simulink model "ekf_pmsm"  (R2026a)
settings: Solver=FixedStepDiscrete  StartTime=0  StopTime=1.5  FixedStep=1/15000
PreLoadFcn:
  | addpath('F:\code\foc\Doc\matlab');
StartFcn:
  | clear sl_if_ctrl sl_ekf sl_pmsm_meas;
libraries: fl_lib x9, nesl_utility x9, ee_lib x1
Description:
  | ATK-BL57H95D20E：Simscape Electrical PMSM + I/F + EKF
settings Model: Creator=15403  LastModifiedBy=15403

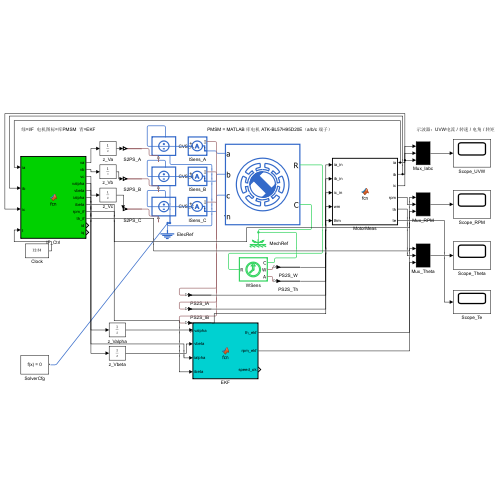
[thumbnail: Simulink's stored preview of the top-level diagram]
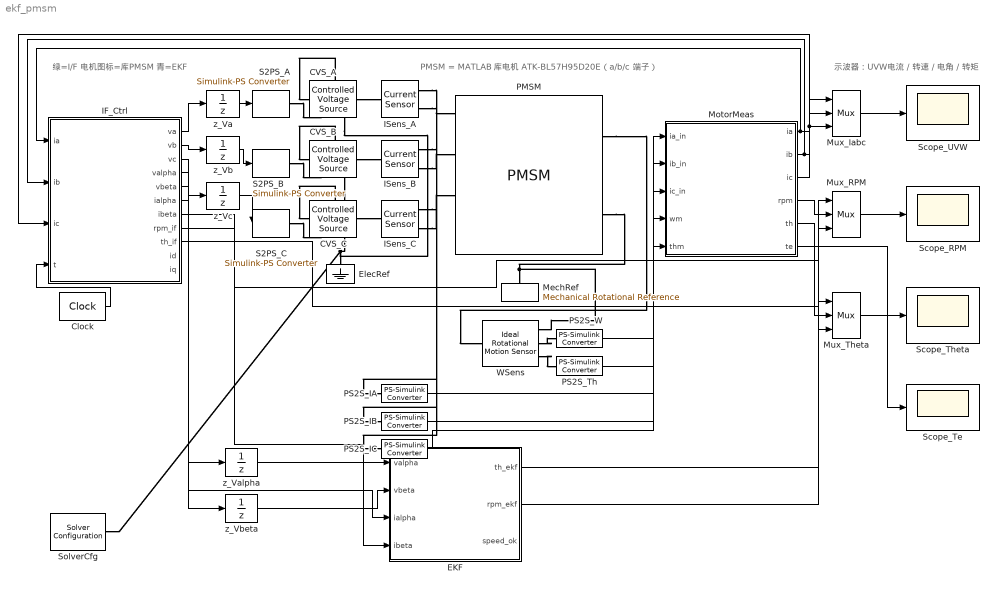
== system ekf_pmsm ==
  note: PMSM = MATLAB 库电机 ATK-BL57H95D20E（a/b/c 端子）
  note: 示波器：UVW电流 / 转速 / 电角 / 转矩
  note: 绿=I/F 电机图标=库PMSM 青=EKF
  CVS_A : fl_lib/Electrical/Electrical Sources/Controlled Voltage Source
  CVS_B : fl_lib/Electrical/Electrical Sources/Controlled Voltage Source
  CVS_C : fl_lib/Electrical/Electrical Sources/Controlled Voltage Source
  Clock : DigitalClock  SampleTime=1/15000
  EKF : MATLAB Function  TreatAsAtomicUnit=on
  ElecRef : fl_lib/Electrical/Electrical Elements/Electrical Reference
  IF_Ctrl : MATLAB Function  TreatAsAtomicUnit=on
  ISens_A : fl_lib/Electrical/Electrical Sensors/Current Sensor
  ISens_B : fl_lib/Electrical/Electrical Sensors/Current Sensor
  ISens_C : fl_lib/Electrical/Electrical Sensors/Current Sensor
  MechRef : fl_lib/Mechanical/Rotational Elements/Mechanical Rotational Reference
  MotorMeas : MATLAB Function  TreatAsAtomicUnit=on
  Mux_Iabc : Mux  Inputs=3
  Mux_RPM : Mux  Inputs=3
  Mux_Theta : Mux  Inputs=3
  PMSM : ee_lib/Electromechanical/Permanent Magnet/PMSM  port_option=ee.enum.threePhasePort.expanded  winding_type=ee.enum.electromech.statorconfiguration.wye  machine_param=ee.enum.pmsm.parameterization.constant  nPolePairs=2  pmflux_param=ee.enum.pmflux.fluxlinkage  pm_flux_linkage=0.02573 Wb  torque_constant=0.18 N*m/A  back_emf_constant=0.18 V*s/rad  stator_param=ee.enum.statorparam.LdLqL0  Ld=0.0008 H  Lq=0.0008 H  idVec=[-200, 0, 200] A  iqVec=[-200, 0, 200] A  LdMatrix=0.0002 * ones(3, 3) H  LqMatrix=0.0002 * ones(3, 3) H  PmMatrix=0.1 * ones(3, 3) Wb  ktMatrix=0.18 * ones(3, 3) N*m/A  keMatrix=0.18 * ones(3, 3) V*s/rad  L0=0.0008 H  Ls=0.0002 H  Lm=-0.00002 H  Ms=0.00002 H  Rs=0.4 Ohm  zero_sequence=ee.enum.park.zerosequence.include  axes_param=ee.enum.rotorangle.daxis  loss_param=ee.enum.ironloss.none  losses_oc=[0, 0, 0] W  losses_sc=[0, 0, 0] W  f_losses=60 Hz  Isc_losses=95 A  J=2.1e-05 kg*m^2  lam=5.25e-05 N*m*s/rad  i_d_specify=off  i_d_priority=None  i_d=0 A  i_d_nominal_specify=off  i_d_nominal_value=1  i_d_nominal_unit=A  i_q_specify=off  i_q_priority=None  i_q=0 A  i_q_nominal_specify=off  i_q_nominal_value=1  i_q_nominal_unit=A  torque_specify=off  torque_priority=None  torque=0 N*m  torque_nominal_specify=off  torque_nominal_value=1  torque_nominal_unit=N*m  angular_velocity_specify=off  angular_velocity_priority=High  angular_velocity=0 rpm  angular_velocity_nominal_specify=off  angular_velocity_nominal_value=1  angular_velocity_nominal_unit=rpm  angular_position_specify=off  angular_position_priority=High  angular_position=0 deg  angular_position_nominal_specify=off  angular_position_nominal_value=1  angular_position_nominal_unit=deg  alpha=3.93e-3 1/K  alpha_flux=-0.001 1/K  Tmeas=298.15 K  stator_thermal_mass=100 J/K  rotor_thermal_mass=200 J/K  Rm_percent_rotor=90  Rd_percent_rotor=30  temperatureA_specify=off  temperatureA_priority=High  temperatureA=25 degC  temperatureA_nominal_specify=off  temperatureA_nominal_value=1  temperatureA_nominal_unit=degC  temperatureB_specify=off  temperatureB_priority=High  temperatureB=25 degC  temperatureB_nominal_specify=off  temperatureB_nominal_value=1  temperatureB_nominal_unit=degC  temperatureC_specify=off  temperatureC_priority=High  temperatureC=25 degC  temperatureC_nominal_specify=off  temperatureC_nominal_value=1  temperatureC_nominal_unit=degC  temperatureR_specify=off  temperatureR_priority=High  temperatureR=25 degC  temperatureR_nominal_specify=off  temperatureR_nominal_value=1  temperatureR_nominal_unit=degC
  PS2S_IA : nesl_utility/PS-Simulink Converter  PhysicalDomain=network_engine_domain  SubClassName=ps_output  LeftPortType=input  RightPortType=output  PseudoPeriodic=off  Frequencies=[]  VectorFormat=inherit  Unit=A  AffineConversion=off
  PS2S_IB : nesl_utility/PS-Simulink Converter  PhysicalDomain=network_engine_domain  SubClassName=ps_output  LeftPortType=input  RightPortType=output  PseudoPeriodic=off  Frequencies=[]  VectorFormat=inherit  Unit=A  AffineConversion=off
  PS2S_IC : nesl_utility/PS-Simulink Converter  PhysicalDomain=network_engine_domain  SubClassName=ps_output  LeftPortType=input  RightPortType=output  PseudoPeriodic=off  Frequencies=[]  VectorFormat=inherit  Unit=A  AffineConversion=off
  PS2S_Th : nesl_utility/PS-Simulink Converter  PhysicalDomain=network_engine_domain  SubClassName=ps_output  LeftPortType=input  RightPortType=output  PseudoPeriodic=off  Frequencies=[]  VectorFormat=inherit  Unit=rad  AffineConversion=off
  PS2S_W : nesl_utility/PS-Simulink Converter  PhysicalDomain=network_engine_domain  SubClassName=ps_output  LeftPortType=input  RightPortType=output  PseudoPeriodic=off  Frequencies=[]  VectorFormat=inherit  Unit=rad/s  AffineConversion=off
  S2PS_A : nesl_utility/Simulink-PS Converter  PhysicalDomain=network_engine_domain  SubClassName=ps_input  LeftPortType=input  RightPortType=output  PseudoPeriodic=off  Frequencies=[]  NoiseDistribution=none  NoiseParameters=[]  Unit=V  AffineConversion=off  FilteringAndDerivatives=provide  SimscapeFilterOrder=1  InputFilterTimeConstant=0.001  UdotUserProvided=0
  S2PS_B : nesl_utility/Simulink-PS Converter  PhysicalDomain=network_engine_domain  SubClassName=ps_input  LeftPortType=input  RightPortType=output  PseudoPeriodic=off  Frequencies=[]  NoiseDistribution=none  NoiseParameters=[]  Unit=V  AffineConversion=off  FilteringAndDerivatives=provide  SimscapeFilterOrder=1  InputFilterTimeConstant=0.001  UdotUserProvided=0
  S2PS_C : nesl_utility/Simulink-PS Converter  PhysicalDomain=network_engine_domain  SubClassName=ps_input  LeftPortType=input  RightPortType=output  PseudoPeriodic=off  Frequencies=[]  NoiseDistribution=none  NoiseParameters=[]  Unit=V  AffineConversion=off  FilteringAndDerivatives=provide  SimscapeFilterOrder=1  InputFilterTimeConstant=0.001  UdotUserProvided=0
  Scope_RPM : Scope
      settings: ActiveDisplayYMinimum=-279.72806706103518  ActiveDisplayYMaximum=2774.0694522575918
  Scope_Te : Scope
      settings: ActiveDisplayYMinimum=-0.00580393372239108  ActiveDisplayYMaximum=0.010794712886261914
  Scope_Theta : Scope
      settings: ActiveDisplayYMinimum=7346.49671423804  ActiveDisplayYMaximum=7512.2082843471344
  Scope_UVW : Scope
      settings: ActiveDisplayYMinimum=-5.0946492100882974  ActiveDisplayYMaximum=4.6567988178636437
  SolverCfg : nesl_utility/Solver Configuration  PhysicalDomain=network_engine_domain  SubClassName=solver  LeftPortType=input  RightPortType=generic  Tones=[]  Harmonics=[]  SimulateNoise=off  Profile=off  UseLocalSampling=off  EnableSwitchedLinearOptims=on  FrequencyDomain=off  UseCCode=off  RelTol=0.001  AbsTol=0.001  MinStep=1e-09  ToWorkspace=off  RevertToSquareIcSolve=off  NumHomotopyIterations=100  PhasorMode=off  PhasorModeNumHarmonics=1  ConsistencySolver=NEWTON_XTOL_AFTER_FTOL  CanonicalOrdering=CANONICAL  OptimizeIntermediates=OPTIMIZED  IndexReductionMethod=DerivativeReplacement  DoDC=off  ResidualTolerance=1e-09  ConsistencyTolSource=GLOBAL  ConsistencyAbsTol=0.001  ConsistencyRelTol=0.001  ConsistencyTolFactor=0.001  UseLocalSolver=on  LocalSolverChoice=NE_BACKWARD_EULER_ADVANCER  ResolveIndetEquations=on  FunctionEvalNumThread=1  LocalSolverSampleTime=1/15000  DoFixedCost=off  MaxNonlinIter=3  MaxModeIter=2  ComputeImpulses=off  ImpulseIterations=2  LinearAlgebra=auto  LinearAlgebraNumThread=0  EquationFormulation=NE_TIME_EF  DelaysMemoryBudget=1024  AutomaticFiltering=on  FilteringTimeConstant=0.001  PartitionStorageMethod=AS_NEEDED  PartitionMemoryBudget=1024  PartitionMethod=ROBUST  MultibodyUseLocalSolver=off  MultibodyLocalSolverChoice=ODE1  MultibodyLocalSolverSampleTime=0.001
  WSens : fl_lib/Mechanical/Mechanical Sensors/Ideal Rotational Motion Sensor  reference=foundation.enum.MeasurementReference.difference  acceleration_port=false  velocity_port=true  position_port=true  wrap_angle=false  offset=0 rad
  z_Va : UnitDelay  SampleTime=1/15000
  z_Valpha : UnitDelay  SampleTime=1/15000
  z_Vb : UnitDelay  SampleTime=1/15000
  z_Vbeta : UnitDelay  SampleTime=1/15000
  z_Vc : UnitDelay  SampleTime=1/15000
  wires:
  Clock/1 -> IF_Ctrl/4(t)
  IF_Ctrl/1(va) -> z_Va/1
  IF_Ctrl/2(vb) -> z_Vb/1
  IF_Ctrl/3(vc) -> z_Vc/1
  IF_Ctrl/4(valpha) -> z_Valpha/1
  IF_Ctrl/5(vbeta) -> z_Vbeta/1
  z_Va/1 -> S2PS_A/1
  z_Vb/1 -> S2PS_B/1
  z_Vc/1 -> S2PS_C/1
  z_Valpha/1 -> EKF/1(valpha)
  z_Vbeta/1 -> EKF/2(vbeta)
  PS2S_IA/1 -> MotorMeas/1(ia_in)
  PS2S_IB/1 -> MotorMeas/2(ib_in)
  PS2S_IC/1 -> MotorMeas/3(ic_in)
  PS2S_W/1 -> MotorMeas/4(wm)
  PS2S_Th/1 -> MotorMeas/5(thm)
  MotorMeas/1(ia) -> IF_Ctrl/1(ia), Mux_Iabc/1
  MotorMeas/2(ib) -> IF_Ctrl/2(ib), Mux_Iabc/2
  MotorMeas/3(ic) -> IF_Ctrl/3(ic), Mux_Iabc/3
  IF_Ctrl/6(ialpha) -> EKF/3(ialpha)
  IF_Ctrl/7(ibeta) -> EKF/4(ibeta)
  IF_Ctrl/8(rpm_if) -> Mux_RPM/1
  MotorMeas/4(rpm) -> Mux_RPM/2
  EKF/2(rpm_ekf) -> Mux_RPM/3
  IF_Ctrl/9(th_if) -> Mux_Theta/1
  MotorMeas/5(th) -> Mux_Theta/2
  EKF/1(th_ekf) -> Mux_Theta/3
  Mux_Iabc/1 -> Scope_UVW/1
  Mux_RPM/1 -> Scope_RPM/1
  Mux_Theta/1 -> Scope_Theta/1
  MotorMeas/6(te) -> Scope_Te/1
  connections:
  CVS_A/LConn1 -- ISens_A/LConn1
  CVS_B/LConn1 -- ISens_B/LConn1
  CVS_C/LConn1 -- ISens_C/LConn1
  ISens_A/RConn2 -- PMSM/LConn1
  ISens_B/RConn2 -- PMSM/LConn2
  ISens_C/RConn2 -- PMSM/LConn3
  CVS_A/RConn2 -- CVS_C/RConn2 -- CVS_B/RConn2 -- ElecRef/LConn1 -- SolverCfg/RConn1
  MechRef/LConn1 -- PMSM/RConn2 -- WSens/RConn1
  PMSM/RConn1 -- WSens/LConn1
  S2PS_A/RConn1 -- CVS_A/RConn1
  S2PS_B/RConn1 -- CVS_B/RConn1
  S2PS_C/RConn1 -- CVS_C/RConn1
  ISens_A/RConn1 -- PS2S_IA/LConn1
  ISens_B/RConn1 -- PS2S_IB/LConn1
  ISens_C/RConn1 -- PS2S_IC/LConn1
  WSens/RConn2 -- PS2S_W/LConn1
  WSens/RConn3 -- PS2S_Th/LConn1

== matlab function ekf_pmsm/MotorMeas ==
  data: ia_in input; ia output; ib_in input; ic_in input; wm input; thm input; ib output; ic output; rpm output; th output; te output
function [ia,ib,ic,rpm,th,te] = fcn(ia_in,ib_in,ic_in,wm,thm)
[ia,ib,ic,rpm,th,te] = sl_pmsm_meas(ia_in,ib_in,ic_in,wm,thm);
end

== matlab function ekf_pmsm/IF_Ctrl ==
  data: ia input; va output; ib input; ic input; t input; vb output; vc output; valpha output; vbeta output; ialpha output; ibeta output; rpm_if output; th_if output; id output; iq output
function [va,vb,vc,valpha,vbeta,ialpha,ibeta,rpm_if,th_if,id,iq] = fcn(ia,ib,ic,t)
[va,vb,vc,valpha,vbeta,ialpha,ibeta,rpm_if,th_if,id,iq] = sl_if_ctrl(ia,ib,ic,t);
end

== matlab function ekf_pmsm/EKF ==
  data: valpha input; th_ekf output; vbeta input; ialpha input; ibeta input; rpm_ekf output; speed_ok output
function [th_ekf,rpm_ekf,speed_ok] = fcn(valpha,vbeta,ialpha,ibeta)
[th_ekf,rpm_ekf,speed_ok] = sl_ekf(valpha,vbeta,ialpha,ibeta);
end
